simulink model "TV_FLC_V3_Codegen"  (R2026a)
settings: Solver=FixedStepDiscrete  StopTime=100  FixedStep=0.003  MaxStep=0.4  AbsTol=1e-3
model workspace (MAT data in the model file):
  Af = 1.20000004768
  C_alpha_F = 46504
  D = 11
  F = 0.0421790704131
  FIS_DYC_3 : fistree (value not decoded)
  Gain = 0.175131350756
  Gr = 5
  I = 6000
  Kp_TV_Beta = Simulink.Parameter
  Kp_TV_Beta.Value = 600
  Kp_TV_Beta.Complexity = 'real'
  Kp_TV_Beta.Dimensions = [1 1]
  Kp_TV_Beta.CoderInfo.StorageClass = 'ImportedExtern'
  Kp_TV_Beta.DataType = 'single'
  Kp_TV_Yaw = Simulink.Parameter
  Kp_TV_Yaw.Value = 1000
  Kp_TV_Yaw.Complexity = 'real'
  Kp_TV_Yaw.Dimensions = [1 1]
  Kp_TV_Yaw.CoderInfo.StorageClass = 'ImportedExtern'
  Kp_TV_Yaw.DataType = 'single'
  Ku = -0.000124337399029
  L = 1.57799994946
  Load_Ref = [0; 400; 500; 600; 700; 800; 900; 1000; 1100; 1200; 1300; 1400; 1500; 1600; 1700; 1800; 1900; 2000]
  MotorT = [51.0306892395 51.0306892395 51.0306892395 51.0306892395 51.0306892395 51.0306892395 51.0306892395 51.0306892395 51.0306892395 51.0306892395 51.0306892395 51.0306892395 51.0306892395 51.0306892395 51.0306892395 51.0306892395 51.0306892395 51.0306892395 51.0306892395 51.0306892395 51.0306892395 51.0306892395 51.0306892395 51.0306892395 51.0306892395 51.0306892395 51.0306892395 51.0306892395 51.0306892395 51.0306892395 51.0306892395 51.0306892395 51.0306892395 51.0306892395 51.0306892395 51.0306892395 51.0306892395 44.8436889648 36.8215675354 30.0627288818 25.3370742798 21.0374126434 17.0840320587 13.4184885025 9.99592685699 6.7769651413 3.73957490921]
  MotorW = [0 100 200 300 400 500 600 700 800 900 1000 1100 1200 1300 1400 1500 1600 1700 1800 1900 2000 2100 2200 2300 2400 2500 2600 2700 2800 2900 3000 3100 3200 3300 3400 3500 3600 3700 3800 3900 4000 4100 4200 4300 4400 4500 4600]
  P = 800
  Slip_Ctrl_Kd = Simulink.Parameter
  Slip_Ctrl_Kd.Value = 0.5
  Slip_Ctrl_Kd.Complexity = 'real'
  Slip_Ctrl_Kd.Dimensions = [1 1]
  Slip_Ctrl_Kd.CoderInfo.StorageClass = 'ImportedExtern'
  Slip_Ctrl_Kd.DataType = 'single'
  Slip_Ctrl_Ki = Simulink.Parameter
  Slip_Ctrl_Ki.Value = 100
  Slip_Ctrl_Ki.Complexity = 'real'
  Slip_Ctrl_Ki.Dimensions = [1 1]
  Slip_Ctrl_Ki.CoderInfo.StorageClass = 'ImportedExtern'
  Slip_Ctrl_Ki.DataType = 'single'
  Slip_Ctrl_Kn = Simulink.Parameter
  Slip_Ctrl_Kn.Value = 100
  Slip_Ctrl_Kn.Complexity = 'real'
  Slip_Ctrl_Kn.Dimensions = [1 1]
  Slip_Ctrl_Kn.CoderInfo.StorageClass = 'ImportedExtern'
  Slip_Ctrl_Kn.DataType = 'single'
  Slip_Ctrl_Kp = Simulink.Parameter
  Slip_Ctrl_Kp.Value = 90
  Slip_Ctrl_Kp.Complexity = 'real'
  Slip_Ctrl_Kp.Dimensions = [1 1]
  Slip_Ctrl_Kp.CoderInfo.StorageClass = 'ImportedExtern'
  Slip_Ctrl_Kp.DataType = 'single'
  Slip_Ref = [0.151999995112; 0.151999995112; 0.151999995112; 0.115999996662; 0.101999998093; 0.0960000008345; 0.0920000001788; 0.0900000035763; 0.0900000035763; 0.0900000035763; 0.0939999967813; 0.097999997437; 0.104000002146; 0.112000003457; 0.126000002027; 0.153999999166; 0.231999993324; 0.15000000596]
  Slip_Steer_th = Simulink.Parameter
  Slip_Steer_th.Value = 15
  Slip_Steer_th.Complexity = 'real'
  Slip_Steer_th.Dimensions = [1 1]
  Slip_Steer_th.CoderInfo.StorageClass = 'ImportedExtern'
  Slip_Steer_th.DataType = 'single'
  Slip_TC_Enable = Simulink.Parameter
  Slip_TC_Enable.Value = 1
  Slip_TC_Enable.Complexity = 'real'
  Slip_TC_Enable.Dimensions = [1 1]
  Slip_TC_Enable.CoderInfo.StorageClass = 'ImportedExtern'
  Slip_TC_Enable.DataType = 'single'
  Tmax = 51.0306892395
  a = 0.823199987411
  a_cop = 0.707000017166
  cd = -2.15000009537
  g = 9.81000041962
  h_CG = 0.358300000429
  m = 320
  ro = 1.22599995136
  rwheel = 0.263000011444
  tr = 1.24800002575
  vx_th = 1
undefined symbols (not defined in the file or in its folder): dspblkCoreblockFVToolHelper, gcbh
libraries: simulink x5, sl_discontinuities x3, slpidlib x2, fuzblock x1
(part 1 of 2)
settings Model: DataDictionary=TV_FLC_V3_Codegen_BusDefs.sldd  Creator=smiller  LastModifiedBy=andrei
settings SolverCC: MaxConsecutiveMinStep=5  InsertRTBMode=Never (minimum delay)  MinimalZcImpactIntegration=on
settings DataIOCC: SaveFormat=StructureWithTime  SignalLoggingName=logsout_sm_car
settings OptimizationCC: UseDivisionForNetSlopeComputation=on  GainParamInheritBuiltInType=on  UseFloatMulNetSlope=on  DefaultUnderspecifiedDataType=single  UseSpecifiedMinMax=on  NoFixptDivByZeroProtection=on  EfficientFloat2IntCast=on
settings DebuggingCC: ReadBeforeWriteMsg=EnableAllAsError  WriteAfterWriteMsg=EnableAllAsError  WriteAfterReadMsg=EnableAllAsError  IntegerOverflowMsg=error  ParameterPrecisionLossMsg=none  UniqueDataStoreMsg=error  NonBusSignalsTreatedAsBus=error  SFInvalidInputDataAccessInChartInitDiag=error  SFTransitionOutsideNaturalParentDiag=error  SFUnreachableExecutionPathDiag=error  SFUndirectedBroadcastEventsDiag=error  IntegerSaturationMsg=error
settings HardwareCC: ProdLargestAtomicInteger=Long  ProdLargestAtomicFloat=Double  ProdHWDeviceType=ARM Compatible->ARM Cortex-M
settings RTWCC: SystemTargetFile=ert.tlc  BuildConfiguration=Faster Runs  Description=Embedded Coder
settings CodeAppCC: CustomSymbolStrGlobalVar=rt$N_$R$M  CustomSymbolStrType=$N_$R$M  CustomSymbolStrFcn=$N$M$F  CustomSymbolStrMacro=$N$M  CustomSymbolStrUtil=$N_$R$C
settings ERTTargetCC: ERTFilePackagingFormat=CompactWithDataFile  GenerateSampleERTMain=on  IncludeMdlTerminateFcn=off  CombineSignalStateStructs=on  SuppressErrorStatus=on  SupportAbsoluteTime=off  CodeInterfacePackaging=Reusable function  SupportComplex=off
settings SimscapeCC: SimscapeNominalValues="[{\"value\":\"1\",\"unit\":\"A\"},{\"value\":\"1\",\"unit\":\"bar\"},{\"value\":\"1\",\"unit\":\"cm^2\"},{\"value\":\"1\",\"unit\":\"cm^3/s\"},{\"value\":\"1\",\"unit\":\"kJ/kg\"},{\"value\":\"1\",\"unit\":\"kW\"},{\"value\":\"1\",\"unit\":\"l\"},{\"value\":\"1\",\"unit\":\"N\"},{\"value\":\"1\",\"unit\":\"N*m\"},{\"value\":\"1\",\"unit\":\"V\"}]"  SimscapeLogSimulationStatistics=on  SimscapeLogName=simlog_sm_car  SimscapeLogDataHistory=100000.0  SimscapeOperatingPoint=ssc_op
settings DiagnosticsConfigSet: SimMechanicsConflictingReferenceFrames=none  SimMechanicsRigidlyBoundBlock=none  SimMechanicsUnsatisfiedHighPriorityTargets=error
settings ExplorerConfigSet: InternalSimMechanicsExplorerSettings="<ExplorerConfiguration><canonicalview>default</canonicalview><AnimationSetting><BasePlaybackSpeed>1.0</BasePlaybackSpeed><PlaybackSpeedFactor>1.0</PlaybackSpeedFactor></AnimationSetting><TilePanel><TileInfo><Tiles Columns=\"1\" Count=\"1\" Rows=\"1\"><Column Weight=\"1\"/><Row Weight=\"1\"/><Tile Height=\"1\" Width=\"1\" X=\"0\" Y=\"0\"/></Tiles></TileInfo><SceneInfo><SceneViewer><BGColor><R>1</R><G>1</G><B>1</B></BGColor><Camera><DoPerspective>on</DoPerspective><Position><X>-22.5734563329168161</X><Y>-2.56079992530625722</Y><Z>1.4393604008155032</Z></Position><Center><X>-23.2962680852000119</X><Y>-1.95845679840359432</Y><Z>1.10064823948317181</Z></Center><Up><X>-0.260205889993916473</X><Y>0.216838241661597014</Y><Z>0.940890042335224552</Z></Up><ViewLimDist>1</ViewLimDist><YLim>0.466307658154998694</YLim><XLim>0.489818968650208741</XLim></Camera></SceneViewer></SceneInfo></TilePanel><MechEditorPanel><Cameras><Camera><Id>Camera1</Id><Value><Name>Track FixO FR</Name><NativeCamera><PositionTrackingFeature>Camera_Frames.Frame_FixO_FR.R</PositionTrackingFeature><CenterTrackingFeature>Camera_Frames.Frame_FixO_FR.R</CenterTrackingFeature><UpVectorTrackingFeature>Camera_Frames.Frame_FixO_FR.R</UpVectorTrackingFeature><CenterTrackingOrigin>off</CenterTrackingOrigin><CenterTrackingDirection>+X</CenterTrackingDirection><UpVectorTrackingDirection>+Z</UpVectorTrackingDirection></NativeCamera></Value></Camera><Camera><Id>Camera2</Id><Value><Name>Track FixO Right</Name><NativeCamera><PositionTrackingFeature>Camera_Frames.Frame_FixO_Right.R</PositionTrackingFeature><CenterTrackingFeature>Camera_Frames.Transform_Camera_Ref.F</CenterTrackingFeature><UpVectorTrackingFeature>Camera_Frames.Frame_FixO_Right.R</UpVectorTrackingFeature><CenterTrackingOrigin>off</CenterTrackingOrigin><CenterTrackingDirection>+Y</CenterTrackingDirection><UpVectorTrackingDirection>+Z</UpVectorTrackingDirection></NativeCamera></Value></Camera><Camera><Id>Camera3</Id><Value><Name>Track FixO RR</Name><NativeCamera><PositionTrackingFeature>Camera_Frames.Frame_FixO_RR.R</PositionTrackingFeature><CenterTrackingFeature>Camera_Frames.Frame_FixO_RR.R</CenterTrackingFeature><UpVectorTrackingFeature>Camera_Frames.Frame_FixO_RR.R</UpVectorTrackingFeature><CenterTrackingOrigin>off</CenterTrackingOrigin><CenterTrackingDirection>+X</CenterTrackingDirection><UpVectorTrackingDirection>+Z</UpVectorTrackingDirection></NativeCamera></Value></Camera><Camera><Id>Camera4</Id><Value><Name>Track FixO RL</Name><NativeCamera><PositionTrackingFeature>Camera_Frames.Frame_FixO_RL.R</PositionTrackingFeature><CenterTrackingFeature>Camera_Frames.Frame_FixO_RL.R</CenterTrackingFeature><UpVectorTrackingFeature>Camera_Frames.Frame_FixO_RL.R</UpVectorTrackingFeature><CenterTrackingOrigin>off</CenterTrackingOrigin><CenterTrackingDirection>+X</CenterTrackingDirection><UpVectorTrackingDirection>+Z</UpVectorTrackingDirection></NativeCamera></Value></Camera><Camera><Id>Camera5</Id><Value><Name>Track FixO Left</Name><NativeCamera><PositionTrackingFeature>Camera_Frames.Frame_FixO_Left.R</PositionTrackingFeature><CenterTrackingFeature>Camera_Frames.Transform_Camera_Ref.F</CenterTrackingFeature><UpVectorTrackingFeature>Camera_Frames.Frame_FixO_Left.R</UpVectorTrackingFeature><CenterTrackingOrigin>off</CenterTrackingOrigin><CenterTrackingDirection>-Y</CenterTrackingDirection><UpVectorTrackingDirection>+Z</UpVectorTrackingDirection></NativeCamera></Value></Camera><Camera><Id>Camera6</Id><Value><Name>Track FixO FL</Name><NativeCamera><PositionTrackingFeature>Camera_Frames.Frame_FixO_FL.R</PositionTrackingFeature><CenterTrackingFeature>Camera_Frames.Frame_FixO_FL.R</CenterTrackingFeature><UpVectorTrackingFeature>Camera_Frames.Frame_FixO_FL.R</UpVectorTrackingFeature><CenterTrackingOrigin>off</CenterTrackingOrigin><CenterTrackingDirection>+X</CenterTrackingDirection><UpVectorTrackingDirection>+Z</UpVectorTrackingDirection></NativeCamera></Value></Camera><Camera><Id>Camera7</Id><Value><Name>Track FixO Top</Name><NativeCamera><PositionTrackingFeature>Camera_Frames.Frame_FixO_Top.R</PositionTrackingFeature><CenterTrackingFeature>Camera_Frames.Frame_FixO_Top.R</CenterTrackingFeature><UpVectorTrackingFeature>Camera_Frames.Frame_FixO_Top.R</UpVectorTrackingFeature><CenterTrackingOrigin>off</CenterTrackingOrigin><CenterTrackingDirection>+X</CenterTrackingDirection><UpVectorTrackingDirection>+Z</UpVectorTrackingDirection></NativeCamera></Value></Camera><Camera><Id>Camera8</Id><Value><Name>Track FixO Front</Name><NativeCamera><PositionTrackingFeature>Camera_Frames.Frame_FixO_Front.R</PositionTrackingFeature><CenterTrackingFeature>Camera_Frames.Frame_FixO_Front.R</CenterTrackingFeature><UpVectorTrackingFeature>Camera_Frames.Frame_FixO_Front.R</UpVectorTrackingFeature><CenterTrackingOrigin>off</CenterTrackingOrigin><CenterTrackingDirection>+X</CenterTrackingDirection><UpVectorTrackingDirection>+Z</UpVectorTrackingDirection></NativeCamera></Value></Camera><Camera><Id>Camera9</Id><Value><Name>Track FixO Rear</Name><NativeCamera><PositionTrackingFeature>Camera_Frames.Frame_FixO_Rear.R</PositionTrackingFeature><CenterTrackingFeature>Camera_Frames.Frame_FixO_Rear.R</CenterTrackingFeature><UpVectorTrackingFeature>Camera_Frames.Frame_FixO_Rear.R</UpVectorTrackingFeature><CenterTrackingOrigin>off</CenterTrackingOrigin><CenterTrackingDirection>+X</CenterTrackingDirection><UpVectorTrackingDirection>+Z</UpVectorTrackingDirection></NativeCamera></Value></Camera><Camera><Id>Camera10</Id><Value><Name>Track FR</Name><NativeCamera><PositionTrackingFeature>Camera_Frames.Frame_FR.R</PositionTrackingFeature><CenterTrackingFeature>Camera_Frames.Frame_FR.R</CenterTrackingFeature><UpVectorTrackingFeature>Camera_Frames.Frame_FR.R</UpVectorTrackingFeature><CenterTrackingOrigin>off</CenterTrackingOrigin><CenterTrackingDirection>+X</CenterTrackingDirection><UpVectorTrackingDirection>+Z</UpVectorTrackingDirection></NativeCamera></Value></Camera><Camera><Id>Camera11</Id><Value><Name>Track Right</Name><NativeCamera><PositionTrackingFeature>Camera_Frames.Frame_Right.R</PositionTrackingFeature><CenterTrackingFeature>Camera_Frames.Transform_Camera_Ref.F</CenterTrackingFeature><UpVectorTrackingFeature>Camera_Frames.Frame_Right.R</UpVectorTrackingFeature><CenterTrackingOrigin>off</CenterTrackingOrigin><CenterTrackingDirection>+Y</CenterTrackingDirection><UpVectorTrackingDirection>+Z</UpVectorTrackingDirection></NativeCamera></Value></Camera><Camera><Id>Camera12</Id><Value><Name>Track RR</Name><NativeCamera><PositionTrackingFeature>Camera_Frames.Frame_RR.R</PositionTrackingFeature><CenterTrackingFeature>Camera_Frames.Frame_RR.R</CenterTrackingFeature><UpVectorTrackingFeature>Camera_Frames.Frame_RR.R</UpVectorTrackingFeature><CenterTrackingOrigin>off</CenterTrackingOrigin><CenterTrackingDirection>+X</CenterTrackingDirection><UpVectorTrackingDirection>+Z</UpVectorTrackingDirection></NativeCamera></Value></Camera><Camera><Id>Camera13</Id><Value><Name>Track RL</Name><NativeCamera><PositionTrackingFeature>Camera_Frames.Frame_RL.R</PositionTrackingFeature><CenterTrackingFeature>Camera_Frames.Frame_RL.R</CenterTrackingFeature><UpVectorTrackingFeature>Camera_Frames.Frame_RL.R</UpVectorTrackingFeature><CenterTrackingOrigin>off</CenterTrackingOrigin><CenterTrackingDirection>+X</CenterTrackingDirection><UpVectorTrackingDirection>+Z</UpVectorTrackingDirection></NativeCamera></Value></Camera><Camera><Id>Camera14</Id><Value><Name>Track Left</Name><NativeCamera><PositionTrackingFeature>Camera_Frames.Frame_Left.R</PositionTrackingFeature><CenterTrackingFeature>Camera_Frames.Transform_Camera_Ref.F</CenterTrackingFeature><UpVectorTrackingFeature>Camera_Frames.Frame_Left.R</UpVectorTrackingFeature><CenterTrackingOrigin>off</CenterTrackingOrigin><CenterTrackingDirection>-Y</CenterTrackingDirection><UpVectorTrackingDirection>+Z</UpVectorTrackingDirection></NativeCamera></Value></Camera><Camera><Id>Camera15</Id><Value><Name>Track FL</Name><NativeCamera><PositionTrackingFeature>Camera_Frames.Frame_FL.R</PositionTrackingFeature><CenterTrackingFeature>Camera_Frames.Frame_FL.R</CenterTrackingFeature><UpVectorTrackingFeature>Camera_Frames.Frame_FL.R</UpVectorTrackingFeature><CenterTrackingOrigin>off</CenterTrackingOrigin><CenterTrackingDirection>+X</CenterTrackingDirection><UpVectorTrackingDirection>+Z</UpVectorTrackingDirection></NativeCamera></Value></Camera><Camera><Id>Camera16</Id><Value><Name>Track Top</Name><NativeCamera><PositionTrackingFeature>Camera_Frames.Frame_Top.R</PositionTrackingFeature><CenterTrackingFeature>Camera_Frames.Frame_Top.R</CenterTrackingFeature><UpVectorTrackingFeature>Camera_Frames.Frame_Top.R</UpVectorTrackingFeature><CenterTrackingOrigin>off</CenterTrackingOrigin><CenterTrackingDirection>+X</CenterTrackingDirection><UpVectorTrackingDirection>+Z</UpVectorTrackingDirection></NativeCamera></Value></Camera><Camera><Id>Camera17</Id><Value><Name>Track Front</Name><NativeCamera><PositionTrackingFeature>Camera_Frames.Frame_Front.R</PositionTrackingFeature><CenterTrackingFeature>Camera_Frames.Frame_Front.R</CenterTrackingFeature><UpVectorTrackingFeature>Camera_Frames.Frame_Front.R</UpVectorTrackingFeature><CenterTrackingOrigin>off</CenterTrackingOrigin><CenterTrackingDirection>+X</CenterTrackingDirection><UpVectorTrackingDirection>+Z</UpVectorTrackingDirection></NativeCamera></Value></Camera><Camera><Id>Camera18</Id><Value><Name>Track Rear</Name><NativeCamera><PositionTrackingFeature>Camera_Frames.Frame_Rear.R</PositionTrackingFeature><CenterTrackingFeature>Camera_Frames.Frame_Rear.R</CenterTrackingFeature><UpVectorTrackingFeature>Camera_Frames.Frame_Rear.R</UpVectorTrackingFeature><CenterTrackingOrigin>off</CenterTrackingOrigin><CenterTrackingDirection>+X</CenterTrackingDirection><UpVectorTrackingDirection>+Z</UpVectorTrackingDirection></NativeCamera></Value></Camera><Camera><Id>Camera19</Id><Value><Name>Track SuspF</Name><NativeCamera><PositionTrackingFeature>Camera_Frames.Frame_SuspF.R</PositionTrackingFeature><CenterTrackingFeature>Camera_Frames.Frame_SuspF.R</CenterTrackingFeature><UpVectorTrackingFeature>Camera_Frames.Frame_SuspF.R</UpVectorTrackingFeature><CenterTrackingOrigin>off</CenterTrackingOrigin><CenterTrackingDirection>+X</CenterTrackingDirection><UpVectorTrackingDirection>+Z</UpVectorTrackingDirection></NativeCamera></Value></Camera><Camera><Id>Camera20</Id><Value><Name>Track SuspR</Name><NativeCamera><PositionTrackingFeature>Camera_Frames.Frame_SuspR.R</PositionTrackingFeature><CenterTrackingFeature>Camera_Frames.Frame_SuspR.R</CenterTrackingFeature><UpVectorTrackingFeature>Camera_Frames.Frame_SuspR.R</UpVectorTrackingFeature><CenterTrackingOrigin>off</CenterTrackingOrigin><CenterTrackingDirection>+X</CenterTrackingDirection><UpVectorTrackingDirection>+Z</UpVectorTrackingDirection></NativeCamera></Value></Camera><Camera><Id>Camera21</Id><Value><Name>Track WheelFR</Name><NativeCamera><PositionTrackingFeature>Camera_Frames.Frame_Wheel_FR.R</PositionTrackingFeature><CenterTrackingFeature>Camera_Frames.Frame_Wheel_FR.R</CenterTrackingFeature><UpVectorTrackingFeature>Camera_Frames.Frame_Wheel_FR.R</UpVectorTrackingFeature><CenterTrackingOrigin>off</CenterTrackingOrigin><CenterTrackingDirection>+X</CenterTrackingDirection><UpVectorTrackingDirection>+Z</UpVectorTrackingDirection></NativeCamera></Value></Camera><Camera><Id>Camera22</Id><Value><Name>Track WheelRR</Name><NativeCamera><PositionTrackingFeature>Camera_Frames.Frame_Wheel_RR.R</PositionTrackingFeature><CenterTrackingFeature>Camera_Frames.Frame_Wheel_RR.R</CenterTrackingFeature><UpVectorTrackingFeature>Camera_Frames.Frame_Wheel_RR.R</UpVectorTrackingFeature><CenterTrackingOrigin>off</CenterTrackingOrigin><CenterTrackingDirection>+X</CenterTrackingDirection><UpVectorTrackingDirection>+Z</UpVectorTrackingDirection></NativeCamera></Value></Camera><Camera><Id>Camera23</Id><Value><Name>Track WheelRL</Name><NativeCamera><PositionTrackingFeature>Camera_Frames.Frame_Wheel_RL.R</PositionTrackingFeature><CenterTrackingFeature>Camera_Frames.Frame_Wheel_RL.R</CenterTrackingFeature><UpVectorTrackingFeature>Camera_Frames.Frame_Wheel_RL.R</UpVectorTrackingFeature><CenterTrackingOrigin>off</CenterTrackingOrigin><CenterTrackingDirection>+X</CenterTrackingDirection><UpVectorTrackingDirection>+Z</UpVectorTrackingDirection></NativeCamera></Value></Camera><Camera><Id>Camera24</Id><Value><Name>Track WheelFL</Name><NativeCamera><PositionTrackingFeature>Camera_Frames.Frame_Wheel_FL.R</PositionTrackingFeature><CenterTrackingFeature>Camera_Frames.Frame_Wheel_FL.R</CenterTrackingFeature><UpVectorTrackingFeature>Camera_Frames.Frame_Wheel_FL.R</UpVectorTrackingFeature><CenterTrackingOrigin>off</CenterTrackingOrigin><CenterTrackingDirection>+X</CenterTrackingDirection><UpVectorTrackingDirection>+Z</UpVectorTrackingDirection></NativeCamera></Value></Camera><Camera><Id>Camera25</Id><Value><Name>View Seat FL</Name><NativeCamera><PositionTrackingFeature>Camera_Frames.Frame_View_Seat_FL.R</PositionTrackingFeature><CenterTrackingFeature>Camera_Frames.Frame_View_Seat_FL.R</CenterTrackingFeature><UpVectorTrackingFeature>Camera_Frames.Frame_View_Seat_FL.R</UpVectorTrackingFeature><CenterTrackingOrigin>off</CenterTrackingOrigin><CenterTrackingDirection>+X</CenterTrackingDirection><UpVectorTrackingDirection>+Z</UpVectorTrackingDirection></NativeCamera></Value></Camera><Camera><Id>Camera26</Id><Value><Name>View Seat FR</Name><NativeCamera><PositionTrackingFeature>Camera_Frames.Frame_View_Seat_FR.R</PositionTrackingFeature><CenterTrackingFeature>Camera_Frames.Frame_View_Seat_FR.R</CenterTrackingFeature><UpVectorTrackingFeature>Camera_Frames.Frame_View_Seat_FR.R</UpVectorTrackingFeature><CenterTrackingOrigin>off</CenterTrackingOrigin><CenterTrackingDirection>+X</CenterTrackingDirection><UpVectorTrackingDirection>+Z</UpVectorTrackingDirection></NativeCamera></Value></Camera><Camera><Id>Camera27</Id><Value><Name>View Susp FR</Name><NativeCamera><PositionTrackingFeature>Camera_Frames.Frame_View_Susp_FR.R</PositionTrackingFeature><CenterTrackingFeature>Camera_Frames.Frame_View_Susp_FR.R</CenterTrackingFeature><UpVectorTrackingFeature>Camera_Frames.Frame_View_Susp_FR.R</UpVectorTrackingFeature><CenterTrackingOrigin>off</CenterTrackingOrigin><CenterTrackingDirection>+X</CenterTrackingDirection><UpVectorTrackingDirection>+Z</UpVectorTrackingDirection></NativeCamera></Value></Camera><Camera><Id>Camera28</Id><Value><Name>View Susp RR</Name><NativeCamera><PositionTrackingFeature>Camera_Frames.Frame_View_Susp_RR.R</PositionTrackingFeature><CenterTrackingFeature>Camera_Frames.Frame_View_Susp_RR.R</CenterTrackingFeature><UpVectorTrackingFeature>Camera_Frames.Frame_View_Susp_RR.R</UpVectorTrackingFeature><CenterTrackingOrigin>off</CenterTrackingOrigin><CenterTrackingDirection>+X</CenterTrackingDirection><UpVectorTrackingDirection>+Z</UpVectorTrackingDirection></NativeCamera></Value></Camera><Camera><Id>Camera29</Id><Value><Name>View Susp RL</Name><NativeCamera><PositionTrackingFeature>Camera_Frames.Frame_View_Susp_RL.R</PositionTrackingFeature><CenterTrackingFeature>Camera_Frames.Frame_View_Susp_RL.R</CenterTrackingFeature><UpVectorTrackingFeature>Camera_Frames.Frame_View_Susp_RL.R</UpVectorTrackingFeature><CenterTrackingOrigin>off</CenterTrackingOrigin><CenterTrackingDirection>+X</CenterTrackingDirection><UpVectorTrackingDirection>+Z</UpVectorTrackingDirection></NativeCamera></Value></Camera><Camera><Id>Camera30</Id><Value><Name>View Susp FL</Name><NativeCamera><PositionTrackingFeature>Camera_Frames.Frame_View_Susp_FL.R</PositionTrackingFeature><CenterTrackingFeature>Camera_Frames.Frame_View_Susp_FL.R</CenterTrackingFeature><UpVectorTrackingFeature>Camera_Frames.Frame_View_Susp_FL.R</UpVectorTrackingFeature><CenterTrackingOrigin>off</CenterTrackingOrigin><CenterTrackingDirection>+X</CenterTrackingDirection><UpVectorTrackingDirection>+Z</UpVectorTrackingDirection></NativeCamera></Value></Camera><Camera><Id>Camera31</Id><Value><Name>Dolly Camera</Name><NativeCamera><PositionTrackingFeature>Camera_Frames.Frame_Dolly.R</PositionTrackingFeature><CenterTrackingFeature>Camera_Frames.Frame_Dolly.R</CenterTrackingFeature><UpVectorTrackingFeature>Camera_Frames.Frame_Dolly.R</UpVectorTrackingFeature><CenterTrackingOrigin>off</CenterTrackingOrigin><CenterTrackingDirection>+X</CenterTrackingDirection><UpVectorTrackingDirection>+Z</UpVectorTrackingDirection></NativeCamera></Value></Camera><Camera><Id>Camera32</Id><Value><Name>Track Dolly Camera</Name><NativeCamera><PositionTrackingFeature>Camera_Frames.Frame_Dolly.R</PositionTrackingFeature><CenterTrackingFeature>Camera_Frames.Transform_Camera_Ref.F</CenterTrackingFeature><UpVectorTrackingFeature>Camera_Frames.World_Frame.W</UpVectorTrackingFeature><CenterTrackingOrigin>on</CenterTrackingOrigin><UpVectorTrackingDirection>+Z</UpVectorTrackingDirection></NativeCamera></Value></Camera></Cameras><GfxPanelCameraMap><MapElement CameraMLId=\"Camera1\" GfxPanelIndex=\"0\"/></GfxPanelCameraMap><VideoCreator><PlaybackSpeedRatio>1.0</PlaybackSpeedRatio><FrameRate>30</FrameRate><VideoFormat>MPEG-4</VideoFormat><FrameSize>[800 450]</FrameSize></VideoCreator></MechEditorPanel></ExplorerConfiguration>"

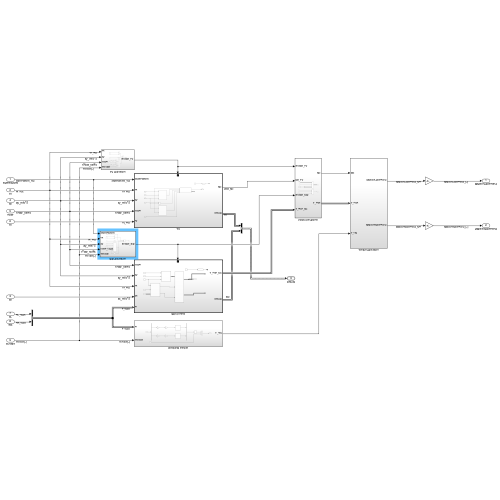
[thumbnail: Simulink's stored preview of the top-level diagram]
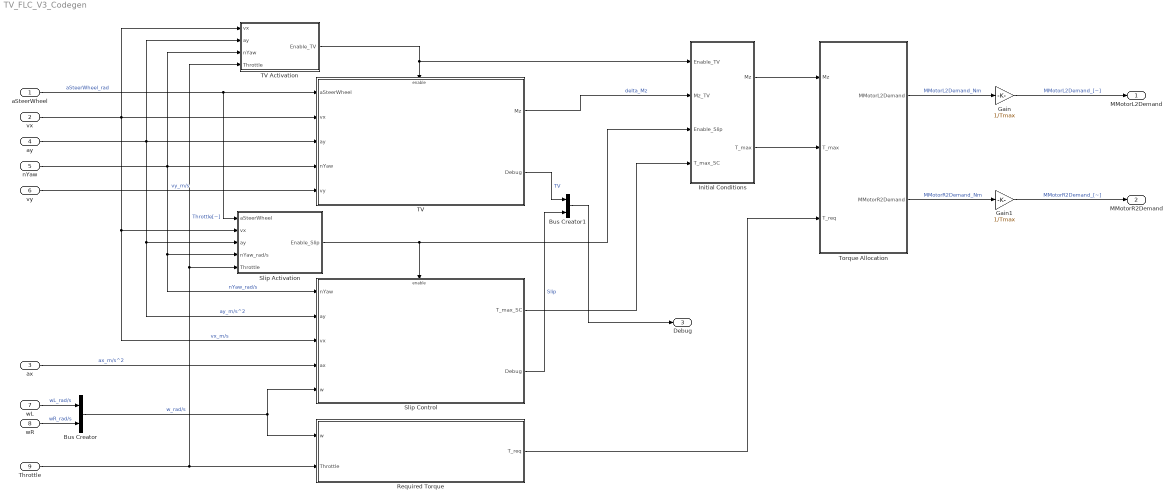
== system TV_FLC_V3_Codegen ==
  aSteerWheel : Inport  OutDataTypeStr=single  PortDimensions=1  SampleTime=0.003
  vx : Inport  Port=2  OutDataTypeStr=single  PortDimensions=1  SampleTime=0.003
  ax : Inport  Port=3  OutDataTypeStr=single  PortDimensions=1  SampleTime=0.003
  ay : Inport  Port=4  OutDataTypeStr=single  PortDimensions=1  SampleTime=0.003
  nYaw : Inport  Port=5  OutDataTypeStr=single  PortDimensions=1  SampleTime=0.003
  vy : Inport  Port=6  OutDataTypeStr=single  PortDimensions=1  SampleTime=0.003
  wL : Inport  Port=7  OutDataTypeStr=single  PortDimensions=1  SampleTime=0.003
  wR : Inport  Port=8  OutDataTypeStr=single  PortDimensions=1  SampleTime=0.003
  Throttle : Inport  Port=9  OutDataTypeStr=single  PortDimensions=1  SampleTime=0.003
  Bus Creator : BusCreator  Inputs=2
  Bus Creator1 : BusCreator  Inputs=2  OutDataTypeStr=Bus: Debug  NonVirtualBus=on
  Gain : Gain  Gain=1/Tmax
  Gain1 : Gain  Gain=1/Tmax
  Initial Conditions : Subsystem
  Required Torque : Subsystem
  Slip Activation : Subsystem
  Slip Control : Subsystem
  TV : Subsystem
  TV Activation : Subsystem
  Torque Allocation : Subsystem
  MMotorL2Demand : Outport  OutDataTypeStr=single  PortDimensions=1  SampleTime=0.003
  MMotorR2Demand : Outport  Port=2  OutDataTypeStr=single  PortDimensions=1  SampleTime=0.003
  Debug : Outport  Port=3  OutDataTypeStr=Bus: Debug  SampleTime=0.003
  wires:
  vy/1 -> TV/5(vy)  "vy_m/s"
  aSteerWheel/1 -> TV/1(aSteerWheel), Slip Activation/1(aSteerWheel)  "aSteerWheel_rad"
  TV/2(Debug) -> Bus Creator1/1  "TV"
  Required Torque/1(T_req) -> Torque Allocation/3(T_req)
  wR/1 -> Bus Creator/2  "wR_rad/s"
  Gain1/1 -> MMotorR2Demand/1  "MMotorR2Demand_[~]"
  TV Activation/1(Enable_TV) -> TV/Enable, Initial Conditions/1(Enable_TV)
  vx/1 -> TV/2(vx), Slip Control/3(vx), Slip Activation/2(vx), TV Activation/1(vx)  "vx_m/s"
  Slip Activation/1(Enable_Slip) -> Initial Conditions/3(Enable_Slip), Slip Control/Enable
  Initial Conditions/2(T_max) -> Torque Allocation/2(T_max)
  ax/1 -> Slip Control/4(ax)  "ax_m/s^2"
  Gain/1 -> MMotorL2Demand/1  "MMotorL2Demand_[~]"
  Slip Control/1(T_max_SC) -> Initial Conditions/4(T_max_SC)
  TV/1(Mz) -> Initial Conditions/2(Mz_TV)  "delta_Mz"
  ay/1 -> TV/3(ay), TV Activation/2(ay), Slip Control/2(ay), Slip Activation/3(ay)  "ay_m/s^2"
  Slip Control/2(Debug) -> Bus Creator1/2  "Slip"
  Initial Conditions/1(Mz) -> Torque Allocation/1(Mz)
  Torque Allocation/1(MMotorL2Demand) -> Gain/1  "MMotorL2Demand_Nm"
  wL/1 -> Bus Creator/1  "wL_rad/s"
  Torque Allocation/2(MMotorR2Demand) -> Gain1/1  "MMotorR2Demand_Nm"
  Bus Creator/1 -> Slip Control/5(w), Required Torque/1(w)  "w_rad/s"
  nYaw/1 -> Slip Control/1(nYaw), Slip Activation/4(nYaw_rad/s), TV/4(nYaw), TV Activation/3(nYaw)  "nYaw_rad/s"
  Throttle/1 -> Required Torque/2(Throttle), Slip Activation/5(Throttle), TV Activation/4(Throttle)  "Throttle[~]"
  Bus Creator1/1 -> Debug/1

== system TV_FLC_V3_Codegen/Initial Conditions ==
  Enable_TV : Inport
  Mz_TV : Inport  Port=2
  Enable_Slip : Inport  Port=3
  T_max_SC : Inport  Port=4
  Bus Creator1 : BusCreator  Inputs=2
  Constant : Constant  Value=Tmax  OutDataTypeStr=single
  Constant1 : Constant  Value=Tmax  OutDataTypeStr=single
  Constant2 : Constant  Value=0  OutDataTypeStr=single
  Switch : Switch  Criteria=u2 ~= 0  SaturateOnIntegerOverflow=off  InputSameDT=off
  Switch1 : Switch  Criteria=u2 ~= 0  SaturateOnIntegerOverflow=off  InputSameDT=off
  Mz : Outport
  T_max : Outport  Port=2
  wires:
  Switch1/1 -> Mz/1
  Constant2/1 -> Switch1/3  "Mz"
  Mz_TV/1 -> Switch1/1
  Constant/1 -> Bus Creator1/1  "Tmax_rl_Nm"
  T_max_SC/1 -> Switch/1
  Bus Creator1/1 -> Switch/3
  Switch/1 -> T_max/1
  Constant1/1 -> Bus Creator1/2  "Tmax_rr_Nm"
  Enable_TV/1 -> Switch1/2
  Enable_Slip/1 -> Switch/2

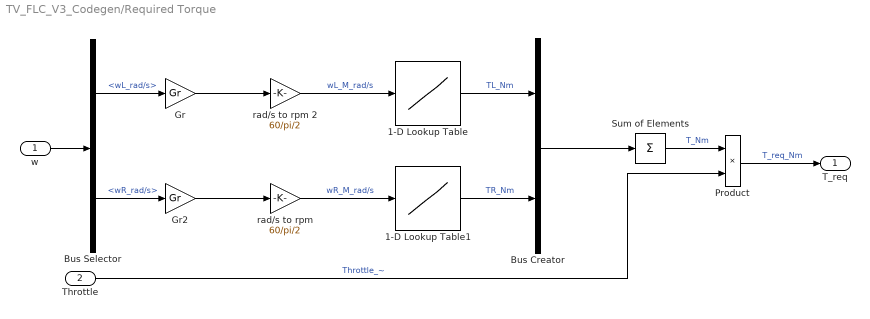
== system TV_FLC_V3_Codegen/Required Torque ==
  w : Inport
  Throttle : Inport  Port=2
  1-D Lookup Table : Lookup_n-D  NumberOfTableDimensions=1  BreakpointsForDimension1=MotorW  Table=MotorT  InternalRulePriority=Speed  RndMeth=Simplest
  1-D Lookup Table1 : Lookup_n-D  NumberOfTableDimensions=1  BreakpointsForDimension1=MotorW  Table=MotorT  InternalRulePriority=Speed  RndMeth=Simplest
  Bus Creator : BusCreator  Inputs=2
  Bus Selector : BusSelector  OutputSignals=wL_rad/s,wR_rad/s
  Gr : Gain  Gain=Gr
  Gr2 : Gain  Gain=Gr
  Product : Product
  Sum of Elements : Sum  Inputs=+
  rad/s to rpm : Gain  Gain=60/pi/2
  rad/s to rpm 2 : Gain  Gain=60/pi/2
  T_req : Outport
  wires:
  Gr2/1 -> rad/s to rpm/1
  Gr/1 -> rad/s to rpm 2/1
  Bus Creator/1 -> Sum of Elements/1
  1-D Lookup Table/1 -> Bus Creator/1  "TL_Nm"
  rad/s to rpm 2/1 -> 1-D Lookup Table/1  "wL_M_rad/s"
  Bus Selector/2 -> Gr2/1  "<wR_rad/s>"
  Product/1 -> T_req/1  "T_req_Nm"
  Bus Selector/1 -> Gr/1  "<wL_rad/s>"
  rad/s to rpm/1 -> 1-D Lookup Table1/1  "wR_M_rad/s"
  Throttle/1 -> Product/2  "Throttle_~"
  1-D Lookup Table1/1 -> Bus Creator/2  "TR_Nm"
  Sum of Elements/1 -> Product/1  "T_Nm"
  w/1 -> Bus Selector/1

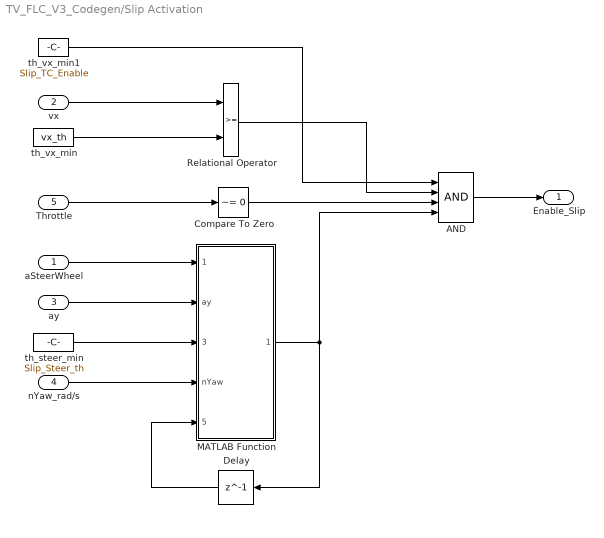
== system TV_FLC_V3_Codegen/Slip Activation ==
  aSteerWheel : Inport
  vx : Inport  Port=2
  ay : Inport  Port=3
  nYaw_rad/s : Inport  Port=4
  Throttle : Inport  Port=5
  AND : Logic  Inputs=4  AllPortsSameDT=off  OutDataTypeStr=boolean
  Compare To Zero : simulink/Logic and Bit Operations/Compare To Zero  relop=~=  OutDataTypeStr=boolean
  Delay : Delay  DelayLength=1
  MATLAB Function : MATLAB Function  TreatAsAtomicUnit=on
  Relational Operator : RelationalOperator  OutDataTypeStr=boolean  RndMeth=Simplest  InputSameDT=off
  th_steer_min : Constant  Value=Slip_Steer_th
  th_vx_min : Constant  Value=vx_th
  th_vx_min1 : Constant  Value=Slip_TC_Enable
  Enable_Slip : Outport
  wires:
  Delay/1 -> MATLAB Function/5(slip_active_previous)
  MATLAB Function/1(slip_active) -> AND/4, Delay/1
  nYaw_rad/s/1 -> MATLAB Function/4(nYaw)
  ay/1 -> MATLAB Function/2(ay)
  th_steer_min/1 -> MATLAB Function/3(steer_th)
  aSteerWheel/1 -> MATLAB Function/1(aSteerWheel)
  Relational Operator/1 -> AND/2
  vx/1 -> Relational Operator/1
  th_vx_min/1 -> Relational Operator/2
  Throttle/1 -> Compare To Zero/1
  AND/1 -> Enable_Slip/1
  Compare To Zero/1 -> AND/3
  th_vx_min1/1 -> AND/1

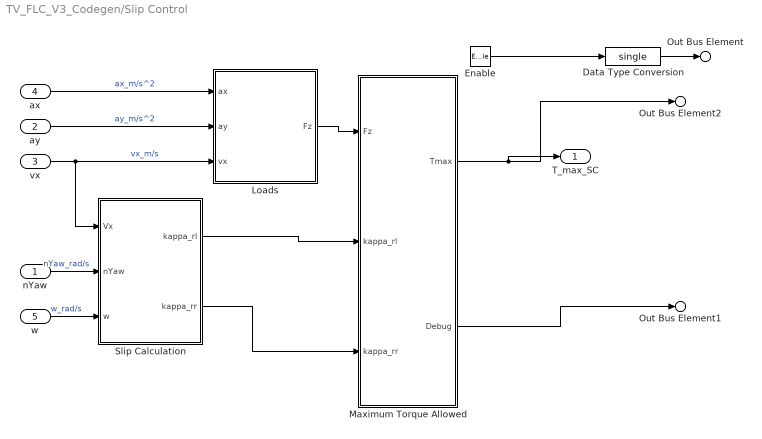
== system TV_FLC_V3_Codegen/Slip Control ==
  nYaw : Inport
  ay : Inport  Port=2
  vx : Inport  Port=3
  ax : Inport  Port=4
  w : Inport  Port=5
  Enable : EnablePort  StatesWhenEnabling=reset  ShowOutputPort=on  OutDataTypeStr=boolean
  Data Type Conversion : DataTypeConversion  OutDataTypeStr=single  SaturateOnIntegerOverflow=off  RndMeth=Floor
  Loads : Subsystem
  Maximum Torque Allowed : Subsystem
  Slip Calculation : Subsystem
  T_max_SC : Outport  OutputWhenDisabled=reset  InitialOutput=Tmax
  Out Bus Element : Outport  Port=2  PortName=Debug  Element=State
  Out Bus Element1 : Outport  Port=2  PortName=Debug  Element=Controller
  Out Bus Element2 : Outport  Port=2  PortName=Debug  Element=TmaxOut
  wires:
  Maximum Torque Allowed/1(Tmax) -> T_max_SC/1, Out Bus Element2/1
  Data Type Conversion/1 -> Out Bus Element/1
  Slip Calculation/1(kappa_rl) -> Maximum Torque Allowed/2(kappa_rl)
  vx/1 -> Slip Calculation/1(Vx), Loads/3(vx)  "vx_m/s"
  Slip Calculation/2(kappa_rr) -> Maximum Torque Allowed/3(kappa_rr)
  ay/1 -> Loads/2(ay)  "ay_m/s^2"
  Loads/1(Fz) -> Maximum Torque Allowed/1(Fz)
  ax/1 -> Loads/1(ax)  "ax_m/s^2"
  nYaw/1 -> Slip Calculation/2(nYaw)  "nYaw_rad/s"
  w/1 -> Slip Calculation/3(w)  "w_rad/s"
  Enable/1 -> Data Type Conversion/1
  Maximum Torque Allowed/2(Debug) -> Out Bus Element1/1

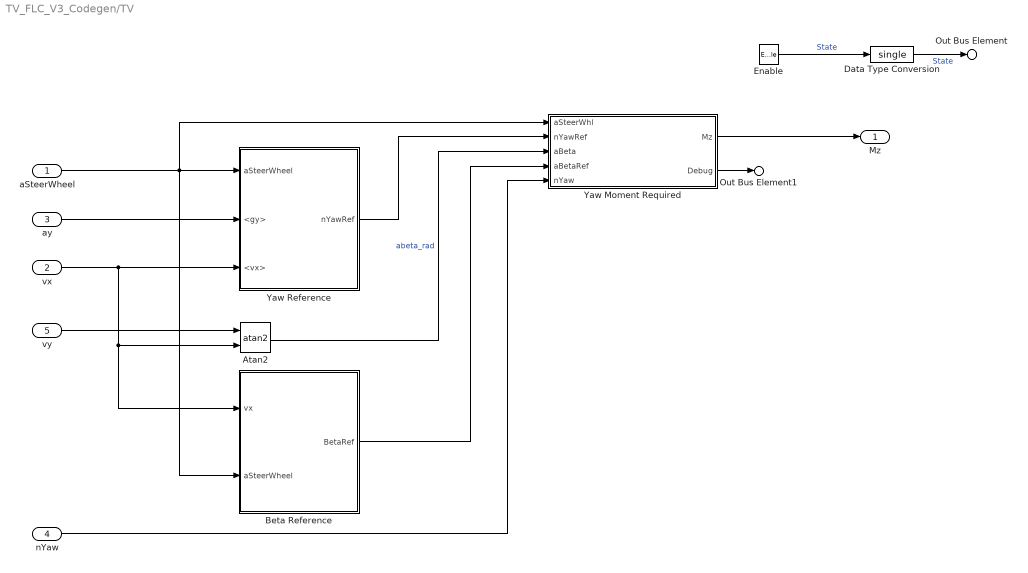
== system TV_FLC_V3_Codegen/TV ==
  aSteerWheel : Inport
  vx : Inport  Port=2
  ay : Inport  Port=3
  nYaw : Inport  Port=4
  vy : Inport  Port=5
  Enable : EnablePort  StatesWhenEnabling=reset  ShowOutputPort=on  OutDataTypeStr=boolean
  Atan2 : Trigonometry  Operator=atan2
  Beta Reference : Subsystem
  Data Type Conversion : DataTypeConversion  OutDataTypeStr=single  SaturateOnIntegerOverflow=off  RndMeth=Floor
  Yaw Moment Required : Subsystem
  Yaw Reference : Subsystem
  Mz : Outport  OutputWhenDisabled=reset  InitialOutput=0
  Out Bus Element : Outport  Port=2  PortName=Debug  Element=State
  Out Bus Element1 : Outport  Port=2  PortName=Debug  Element=Controller
  wires:
  Enable/1 -> Data Type Conversion/1  "State"
  Yaw Moment Required/1(Mz) -> Mz/1
  Atan2/1 -> Yaw Moment Required/3(aBeta)  "abeta_rad"
  aSteerWheel/1 -> Beta Reference/2(aSteerWheel), Yaw Moment Required/1(aSteerWhl), Yaw Reference/1(aSteerWheel)
  vx/1 -> Beta Reference/1(vx), Atan2/2, Yaw Reference/3(<vx>)
  nYaw/1 -> Yaw Moment Required/5(nYaw)
  ay/1 -> Yaw Reference/2(<gy>)
  Yaw Reference/1(nYawRef) -> Yaw Moment Required/2(nYawRef)
  Beta Reference/1(BetaRef) -> Yaw Moment Required/4(aBetaRef)
  vy/1 -> Atan2/1
  Data Type Conversion/1 -> Out Bus Element/1  "State"
  Yaw Moment Required/2(Debug) -> Out Bus Element1/1

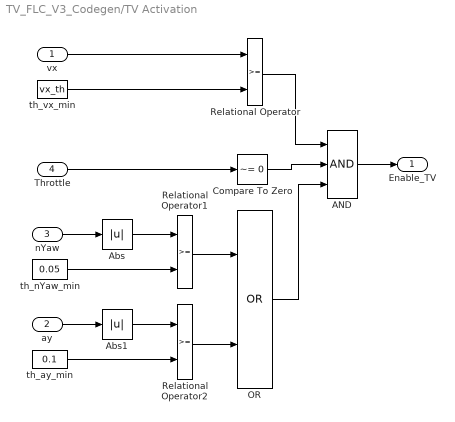
== system TV_FLC_V3_Codegen/TV Activation ==
  vx : Inport
  ay : Inport  Port=2
  nYaw : Inport  Port=3
  Throttle : Inport  Port=4
  AND : Logic  Inputs=3  AllPortsSameDT=off  OutDataTypeStr=boolean
  Abs : Abs  SaturateOnIntegerOverflow=off
  Abs1 : Abs  SaturateOnIntegerOverflow=off
  Compare To Zero : simulink/Logic and Bit Operations/Compare To Zero  relop=~=  OutDataTypeStr=boolean
  OR : Logic  Operator=OR  AllPortsSameDT=off  OutDataTypeStr=boolean
  Relational Operator : RelationalOperator  OutDataTypeStr=boolean  RndMeth=Simplest  InputSameDT=off
  Relational Operator1 : RelationalOperator  OutDataTypeStr=boolean  RndMeth=Simplest  InputSameDT=off
  Relational Operator2 : RelationalOperator  OutDataTypeStr=boolean  RndMeth=Simplest  InputSameDT=off
  th_ay_min : Constant  Value=0.1  OutDataTypeStr=single
  th_nYaw_min : Constant  Value=0.05  OutDataTypeStr=single
  th_vx_min : Constant  Value=vx_th
  Enable_TV : Outport
  wires:
  AND/1 -> Enable_TV/1
  OR/1 -> AND/3
  Compare To Zero/1 -> AND/2
  Relational Operator/1 -> AND/1
  Relational Operator2/1 -> OR/2
  Relational Operator1/1 -> OR/1
  th_vx_min/1 -> Relational Operator/2
  th_ay_min/1 -> Relational Operator2/2
  nYaw/1 -> Abs/1
  vx/1 -> Relational Operator/1
  Abs/1 -> Relational Operator1/1
  Throttle/1 -> Compare To Zero/1
  Abs1/1 -> Relational Operator2/1
  th_nYaw_min/1 -> Relational Operator1/2
  ay/1 -> Abs1/1

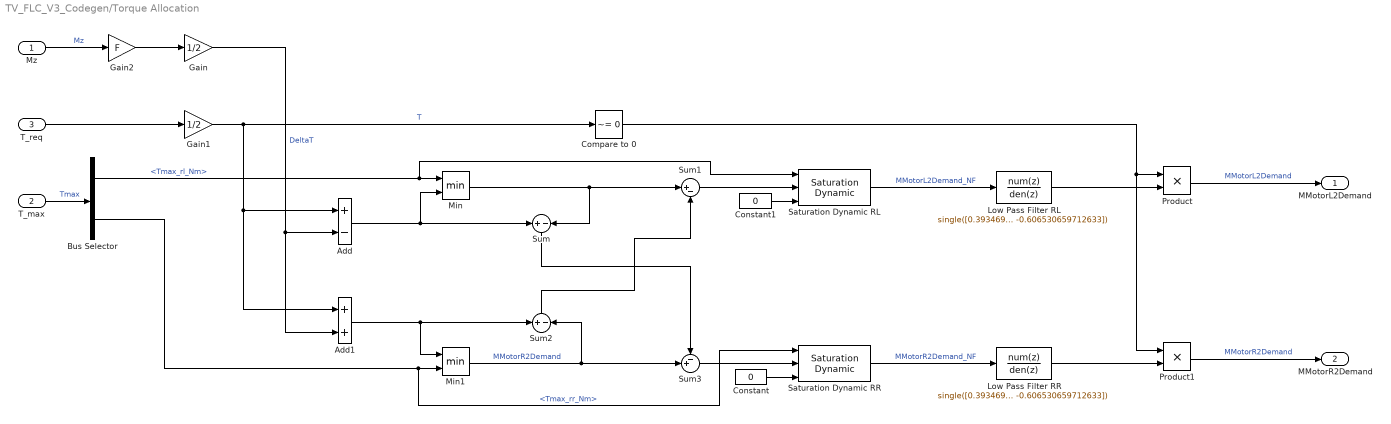
== system TV_FLC_V3_Codegen/Torque Allocation ==
  Mz : Inport
  T_max : Inport  Port=2
  T_req : Inport  Port=3
  Add : Sum  Inputs=+-
  Add1 : Sum
  Bus Selector : BusSelector  OutputSignals=Tmax_rl_Nm,Tmax_rr_Nm
  "Compare to 0 " : simulink/Logic and Bit Operations/Compare To Constant  relop=~=  const=0  OutDataTypeStr=boolean
  Constant : Constant  Value=0
  Constant1 : Constant  Value=0
  Gain : Gain  Gain=1/2
  Gain1 : Gain  Gain=1/2
  Gain2 : Gain  Gain=F
  Low Pass Filter RL : DiscreteTransferFcn  LoadFcn=dspblkCoreblockFVToolHelper(gcbh,'load');  Numerator=single([0.393469340287367])  Denominator=single([1 -0.606530659712633])
      settings: CopyFcn=dspblkCoreblockFVToolHelper(gcbh,'copy');  DeleteFcn=dspblkCoreblockFVToolHelper(gcbh,'close');  ModelCloseFcn=dspblkCoreblockFVToolHelper(gcbh,'close');  PreSaveFcn=dspblkCoreblockFVToolHelper(gcbh,'presave');  PostSaveFcn=dspblkCoreblockFVToolHelper(gcbh,'postsave');  CloseFcn=dspblkCoreblockFVToolHelper(gcbh,'close');
  Low Pass Filter RR : DiscreteTransferFcn  LoadFcn=dspblkCoreblockFVToolHelper(gcbh,'load');  Numerator=single([0.393469340287367])  Denominator=single([1 -0.606530659712633])
      settings: CopyFcn=dspblkCoreblockFVToolHelper(gcbh,'copy');  DeleteFcn=dspblkCoreblockFVToolHelper(gcbh,'close');  ModelCloseFcn=dspblkCoreblockFVToolHelper(gcbh,'close');  PreSaveFcn=dspblkCoreblockFVToolHelper(gcbh,'presave');  PostSaveFcn=dspblkCoreblockFVToolHelper(gcbh,'postsave');  CloseFcn=dspblkCoreblockFVToolHelper(gcbh,'close');
  Min : MinMax  Inputs=2
  Min1 : MinMax  Inputs=2
  Product : Product
  Product1 : Product
  Saturation Dynamic RL : sl_discontinuities/Saturation Dynamic  OutMin=[]  OutMax=[]  OutDataTypeStr=single  OutDataType=fixdt(1, 16)  OutScaling=2^-10  DoSatur=off
      settings: LibrarySourceBlock=|
      | simulink/Discontinuities/Saturation
      | Dynamic
  Saturation Dynamic RR : sl_discontinuities/Saturation Dynamic  OutMin=[]  OutMax=[]  OutDataTypeStr=single  OutDataType=fixdt(1, 16)  OutScaling=2^-10  DoSatur=off
      settings: LibrarySourceBlock=|
      | simulink/Discontinuities/Saturation
      | Dynamic
  Sum : Sum  Inputs=+|-
  Sum1 : Sum  Inputs=|+-
  Sum2 : Sum  Inputs=+|-
  Sum3 : Sum  Inputs=-+|
  MMotorL2Demand : Outport
  MMotorR2Demand : Outport  Port=2
  wires:
  Saturation Dynamic RL/1 -> Low Pass Filter RL/1  "MMotorL2Demand_NF"
  Sum3/1 -> Saturation Dynamic RR/2
  Sum1/1 -> Saturation Dynamic RL/2
  Gain2/1 -> Gain/1
  Gain/1 -> Add1/2, Add/2  "DeltaT"
  T_req/1 -> Gain1/1
  Mz/1 -> Gain2/1  "Mz"
  Min/1 -> Sum1/1, Sum/2
  Min1/1 -> Sum2/2, Sum3/2  "MMotorR2Demand"
  T_max/1 -> Bus Selector/1  "Tmax"
  Bus Selector/1 -> Saturation Dynamic RL/1, Min/1  "<Tmax_rl_Nm>"
  Bus Selector/2 -> Min1/2, Saturation Dynamic RR/1  "<Tmax_rr_Nm>"
  Add/1 -> Sum/1, Min/2
  Add1/1 -> Sum2/1, Min1/1
  Sum2/1 -> Sum1/2
  Sum/1 -> Sum3/1
  Gain1/1 -> "Compare to 0 "/1, Add1/1, Add/1  "T"
  "Compare to 0 "/1 -> Product/1, Product1/1
  Low Pass Filter RL/1 -> Product/2
  Product/1 -> MMotorL2Demand/1  "MMotorL2Demand"
  Saturation Dynamic RR/1 -> Low Pass Filter RR/1  "MMotorR2Demand_NF"
  Low Pass Filter RR/1 -> Product1/2
  Product1/1 -> MMotorR2Demand/1  "MMotorR2Demand"
  Constant/1 -> Saturation Dynamic RR/3
  Constant1/1 -> Saturation Dynamic RL/3

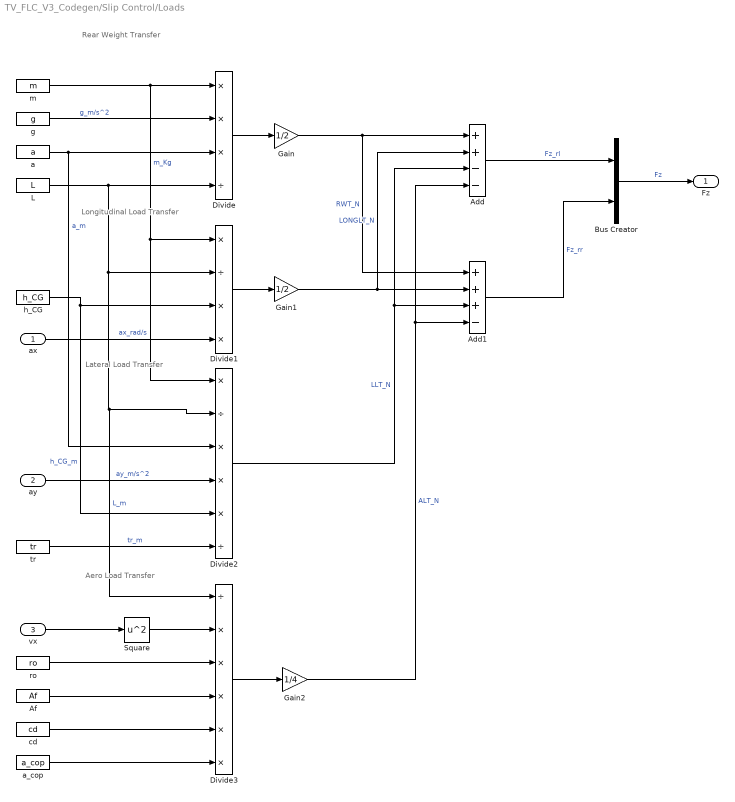
== system TV_FLC_V3_Codegen/Slip Control/Loads ==
  note: Aero Load Transfer
  note: Lateral Load Transfer
  note: Longitudinal Load Transfer
  note: Rear Weight Transfer
  ax : Inport
  ay : Inport  Port=2
  vx : Inport  Port=3
  Add : Sum  Inputs=++--
  Add1 : Sum  Inputs=+++-
  Af : Constant  Value=Af  OutDataTypeStr=single
  Bus Creator : BusCreator  Inputs=2
  Divide : Product  Inputs=***/
  Divide1 : Product  Inputs=*/**
  Divide2 : Product  Inputs=*/***/
  Divide3 : Product  Inputs=/*****
  Gain : Gain  Gain=1/2
  Gain1 : Gain  Gain=1/2
  Gain2 : Gain  Gain=1/4
  L : Constant  Value=L  OutDataTypeStr=single
  Square : Math  Operator=square
  a : Constant  Value=a  OutDataTypeStr=single
  a_cop : Constant  Value=a_cop  OutDataTypeStr=single
  cd : Constant  Value=cd  OutDataTypeStr=single
  g : Constant  Value=g  OutDataTypeStr=single
  h_CG : Constant  Value=h_CG  OutDataTypeStr=single
  m : Constant  Value=m  OutDataTypeStr=single
  ro : Constant  Value=ro  OutDataTypeStr=single
  tr : Constant  Value=tr  OutDataTypeStr=single
  Fz : Outport
  wires:
  m/1 -> Divide/1, Divide1/1, Divide2/1  "m_Kg"
  g/1 -> Divide/2  "g_m/s^2"
  a/1 -> Divide/3, Divide2/3  "a_m"
  L/1 -> Divide3/1, Divide2/2, Divide1/2, Divide/4  "L_m"
  Divide/1 -> Gain/1
  vx/1 -> Square/1
  Square/1 -> Divide3/2
  Gain/1 -> Add/1, Add1/1  "RWT_N"
  Gain2/1 -> Add/4, Add1/4  "ALT_N"
  h_CG/1 -> Divide2/5, Divide1/3  "h_CG_m"
  ax/1 -> Divide1/4  "ax_rad/s"
  Divide1/1 -> Gain1/1
  Gain1/1 -> Add/2, Add1/2  "LONGLT_N"
  ay/1 -> Divide2/4  "ay_m/s^2"
  tr/1 -> Divide2/6  "tr_m"
  Divide2/1 -> Add/3, Add1/3  "LLT_N"
  Add/1 -> Bus Creator/1  "Fz_rl"
  Add1/1 -> Bus Creator/2  "Fz_rr"
  Bus Creator/1 -> Fz/1  "Fz"
  Divide3/1 -> Gain2/1
  ro/1 -> Divide3/3
  Af/1 -> Divide3/4
  cd/1 -> Divide3/5
  a_cop/1 -> Divide3/6

== system TV_FLC_V3_Codegen/Slip Control/Maximum Torque Allowed ==
  Fz : Inport
  kappa_rl : Inport  Port=2
  kappa_rr : Inport  Port=3
  Bus Creator : BusCreator  Inputs=2
  Bus Selector : BusSelector  OutputSignals=Fz_rl,Fz_rr
  Slip Correction Left : Subsystem
  Slip Correction Right : Subsystem
  Tmax : Outport  OutDataTypeStr=single
  Out Bus Element : Outport  Port=2  PortName=Debug  Element=PID_rl
  Out Bus Element1 : Outport  Port=2  PortName=Debug  Element=PID_rr
  wires:
  Bus Creator/1 -> Tmax/1
  Bus Selector/2 -> Slip Correction Right/1(Fz_rl)  "<Fz_rr>"
  Bus Selector/1 -> Slip Correction Left/2(Fz_rl)  "<Fz_rl>"
  Fz/1 -> Bus Selector/1
  kappa_rr/1 -> Slip Correction Right/2(kappa_rr)
  kappa_rl/1 -> Slip Correction Left/1(kappa_rl)
  Slip Correction Left/2(Tmax_rl) -> Bus Creator/1  "Tmax_rl_Nm"
  Slip Correction Right/1(Tmax_rr) -> Bus Creator/2  "Tmax_rr_Nm"
  Slip Correction Left/1(Debug) -> Out Bus Element/1
  Slip Correction Right/2(Debug) -> Out Bus Element1/1

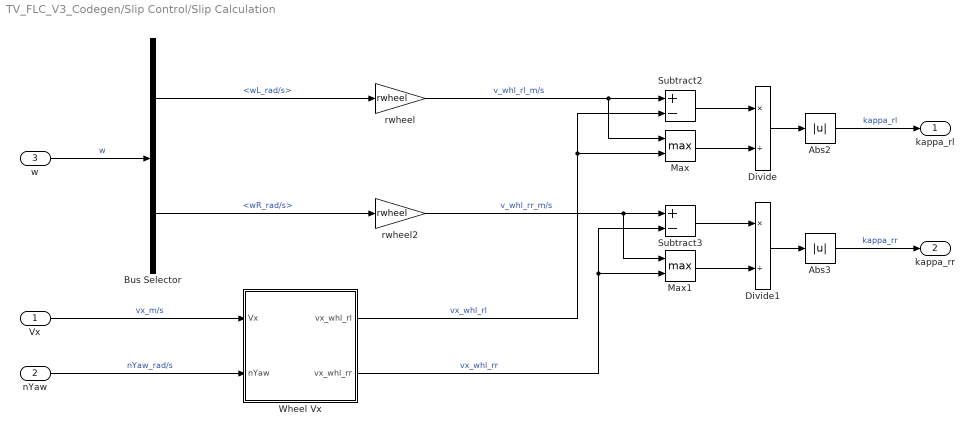
== system TV_FLC_V3_Codegen/Slip Control/Slip Calculation ==
  Vx : Inport
  nYaw : Inport  Port=2
  w : Inport  Port=3
  Abs2 : Abs  SaturateOnIntegerOverflow=off
  Abs3 : Abs  SaturateOnIntegerOverflow=off
  Bus Selector : BusSelector  OutputSignals=wL_rad/s,wR_rad/s
  Divide : Product  Inputs=*/
  Divide1 : Product  Inputs=*/
  Max : MinMax  Function=max  Inputs=2
  Max1 : MinMax  Function=max  Inputs=2
  Subtract2 : Sum  Inputs=+-
  Subtract3 : Sum  Inputs=+-
  Wheel Vx : Subsystem
  rwheel : Gain  Gain=rwheel
  rwheel2 : Gain  Gain=rwheel
  kappa_rl : Outport
  kappa_rr : Outport  Port=2
  wires:
  Bus Selector/1 -> rwheel/1  "<wL_rad/s>"
  Bus Selector/2 -> rwheel2/1  "<wR_rad/s>"
  Vx/1 -> Wheel Vx/1(Vx)  "vx_m/s"
  w/1 -> Bus Selector/1  "w"
  rwheel/1 -> Max/1, Subtract2/1  "v_whl_rl_m/s"
  rwheel2/1 -> Max1/1, Subtract3/1  "v_whl_rr_m/s"
  nYaw/1 -> Wheel Vx/2(nYaw)  "nYaw_rad/s"
  Abs3/1 -> kappa_rr/1  "kappa_rr"
  Wheel Vx/1(vx_whl_rl) -> Subtract2/2, Max/2  "vx_whl_rl"
  Abs2/1 -> kappa_rl/1  "kappa_rl"
  Subtract2/1 -> Divide/1
  Wheel Vx/2(vx_whl_rr) -> Subtract3/2, Max1/2  "vx_whl_rr"
  Subtract3/1 -> Divide1/1
  Divide/1 -> Abs2/1
  Max/1 -> Divide/2
  Divide1/1 -> Abs3/1
  Max1/1 -> Divide1/2

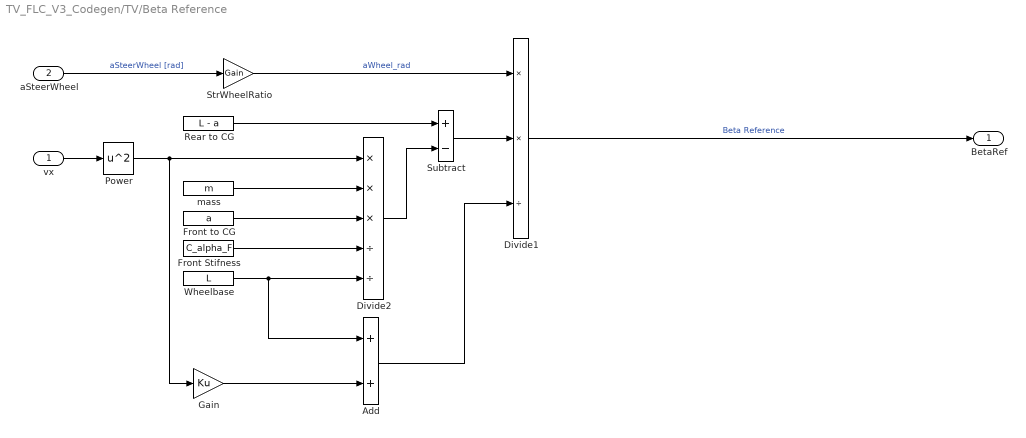
== system TV_FLC_V3_Codegen/TV/Beta Reference ==
  vx : Inport
  aSteerWheel : Inport  Port=2
  Add : Sum
  Divide1 : Product  Inputs=**/
  Divide2 : Product  Inputs=***//
  Front Stifness : Constant  Value=C_alpha_F  OutDataTypeStr=single
  Front to CG : Constant  Value=a  OutDataTypeStr=single
  Gain : Gain  Gain=Ku  ParamDataTypeStr=single
  Power : Math  Operator=square
  Rear to CG : Constant  Value=L - a  OutDataTypeStr=single
  StrWheelRatio : Gain  Gain=Gain
  Subtract : Sum  Inputs=+-
  Wheelbase : Constant  Value=L  OutDataTypeStr=single
  mass : Constant  Value=m  OutDataTypeStr=single
  BetaRef : Outport
  wires:
  StrWheelRatio/1 -> Divide1/1  "aWheel_rad"
  Add/1 -> Divide1/3
  Gain/1 -> Add/2
  Power/1 -> Gain/1, Divide2/1
  Divide1/1 -> BetaRef/1  "Beta Reference"
  vx/1 -> Power/1
  aSteerWheel/1 -> StrWheelRatio/1  "aSteerWheel [rad]"
  Wheelbase/1 -> Add/1, Divide2/5
  Front Stifness/1 -> Divide2/4
  mass/1 -> Divide2/2
  Front to CG/1 -> Divide2/3
  Rear to CG/1 -> Subtract/1
  Divide2/1 -> Subtract/2
  Subtract/1 -> Divide1/2

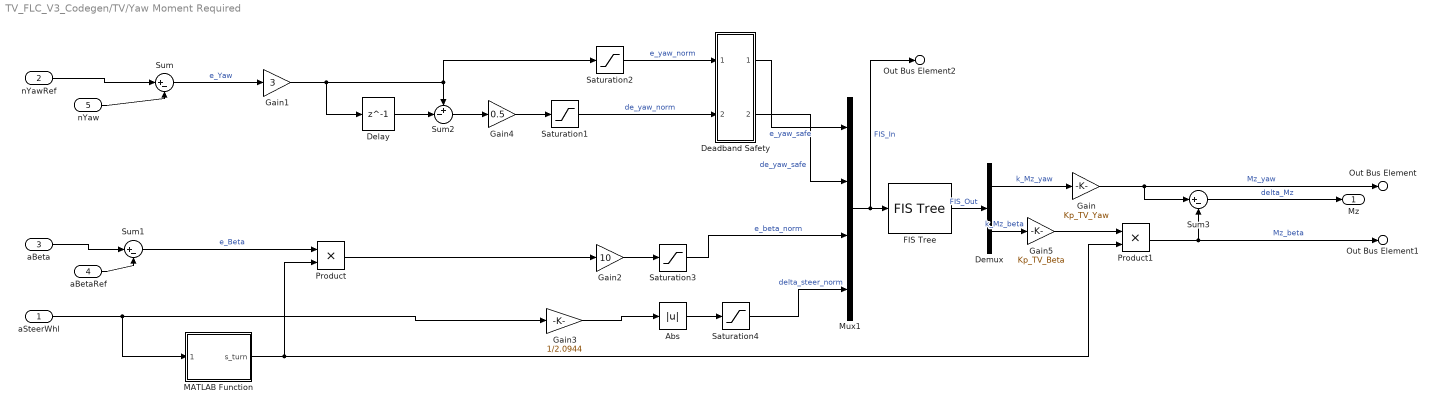
== system TV_FLC_V3_Codegen/TV/Yaw Moment Required ==
  aSteerWhl : Inport  OutDataTypeStr=single
  nYawRef : Inport  Port=2  OutDataTypeStr=single
  aBeta : Inport  Port=3  OutDataTypeStr=single
  aBetaRef : Inport  Port=4  OutDataTypeStr=single
  nYaw : Inport  Port=5  OutDataTypeStr=single
  Abs : Abs  SaturateOnIntegerOverflow=off
  Deadband Safety : Subsystem
  Delay : Delay  DelayLength=1  InputProcessing=Columns as channels (frame based)
  Demux : Demux  Outputs=2
  FIS Tree : fuzblock/FIS Tree  FIS=FIS_DYC_3  OutputSampleNumber=101  DataType=single  SimulateUsing=Code generation  OutOfRangeInputValueMessage=warning  NoRuleFiredMessage=warning  EmptyOutputFuzzySetMessage=warning
  Gain : Gain  Gain=Kp_TV_Yaw  OutDataTypeStr=single
  Gain1 : Gain  Gain=3
  Gain2 : Gain  Gain=10  OutDataTypeStr=single
  Gain3 : Gain  Gain=1/2.0944  OutDataTypeStr=single
  Gain4 : Gain  Gain=0.5
  Gain5 : Gain  Gain=Kp_TV_Beta  OutDataTypeStr=single
  MATLAB Function : MATLAB Function  TreatAsAtomicUnit=on  mask{delta_th=Slip_Steer_th/2}
      mask prompts: delta_th "Steering Th"
  Mux1 : Mux
  Product : Product
  Product1 : Product
  Saturation1 : Saturate  UpperLimit=1  LowerLimit=-1
  Saturation2 : Saturate  UpperLimit=1  LowerLimit=-1
  Saturation3 : Saturate  UpperLimit=1  LowerLimit=-1  ZeroCross=off
  Saturation4 : Saturate  UpperLimit=1  LowerLimit=0  ZeroCross=off
  Sum : Sum  Inputs=|+-
  Sum1 : Sum  Inputs=|+-
  Sum2 : Sum  Inputs=+-|
  Sum3 : Sum  Inputs=|+-  OutDataTypeStr=Inherit: Same as first input
  Mz : Outport  OutDataTypeStr=single
  Out Bus Element : Outport  Port=2  PortName=Debug  Element=Mz_yaw
  Out Bus Element1 : Outport  Port=2  PortName=Debug  Element=Mz_Beta
  Out Bus Element2 : Outport  Port=2  PortName=Debug  Element=FIS_In
  wires:
  Sum/1 -> Gain1/1  "e_Yaw"
  nYaw/1 -> Sum/2
  nYawRef/1 -> Sum/1
  FIS Tree/1 -> Demux/1  "FIS_Out"
  Gain/1 -> Out Bus Element/1, Sum3/1  "Mz_yaw"
  Delay/1 -> Sum2/2
  Sum2/1 -> Gain4/1
  Mux1/1 -> Out Bus Element2/1, FIS Tree/1  "FIS_In"
  Sum1/1 -> Product/1  "e_Beta"
  aBeta/1 -> Sum1/1
  aBetaRef/1 -> Sum1/2
  aSteerWhl/1 -> Gain3/1, MATLAB Function/1(delta_SW)
  Gain1/1 -> Delay/1, Sum2/1, Saturation2/1
  Gain2/1 -> Saturation3/1
  Gain3/1 -> Abs/1
  Saturation3/1 -> Mux1/3  "e_beta_norm"
  Saturation4/1 -> Mux1/4  "delta_steer_norm"
  Gain4/1 -> Saturation1/1
  MATLAB Function/1(s_turn) -> Product/2, Product1/2
  Product/1 -> Gain2/1
  Demux/1 -> Gain/1  "k_Mz_yaw"
  Demux/2 -> Gain5/1  "k_Mz_beta"
  Sum3/1 -> Mz/1  "delta_Mz"
  Gain5/1 -> Product1/1
  Product1/1 -> Out Bus Element1/1, Sum3/2  "Mz_beta"
  Abs/1 -> Saturation4/1
  Saturation2/1 -> Deadband Safety/1(e_yaw_norm)  "e_yaw_norm"
  Saturation1/1 -> Deadband Safety/2(de_yaw_norm)  "de_yaw_norm"
  Deadband Safety/1(e_yaw_safe) -> Mux1/1  "e_yaw_safe"
  Deadband Safety/2(de_yaw_safe) -> Mux1/2  "de_yaw_safe"

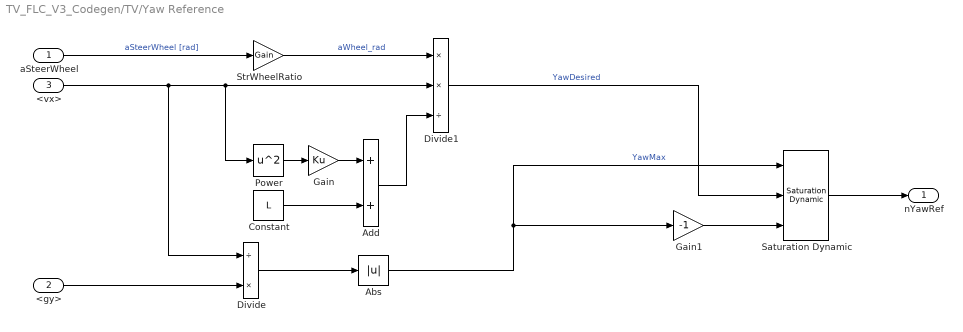
== system TV_FLC_V3_Codegen/TV/Yaw Reference ==
  aSteerWheel : Inport
  <gy> : Inport  Port=2
  <vx> : Inport  Port=3
  Abs : Abs  SaturateOnIntegerOverflow=off
  Add : Sum
  Constant : Constant  Value=L  OutDataTypeStr=single
  Divide : Product  Inputs=/*
  Divide1 : Product  Inputs=**/
  Gain : Gain  Gain=Ku
  Gain1 : Gain  Gain=-1
  Power : Math  Operator=square
  Saturation Dynamic : sl_discontinuities/Saturation Dynamic  OutMin=[]  OutMax=[]  OutDataTypeStr=Inherit: Same as second input  OutDataType=fixdt(1, 16)  OutScaling=2^-10  DoSatur=off
  StrWheelRatio : Gain  Gain=Gain
  nYawRef : Outport
  wires:
  StrWheelRatio/1 -> Divide1/1  "aWheel_rad"
  aSteerWheel/1 -> StrWheelRatio/1  "aSteerWheel [rad]"
  <vx>/1 -> Divide1/2, Power/1, Divide/1
  <gy>/1 -> Divide/2
  Divide/1 -> Abs/1
  Saturation Dynamic/1 -> nYawRef/1
  Abs/1 -> Saturation Dynamic/1, Gain1/1  "YawMax"
  Gain1/1 -> Saturation Dynamic/3
  Divide1/1 -> Saturation Dynamic/2  "YawDesired"
  Power/1 -> Gain/1
  Gain/1 -> Add/1
  Constant/1 -> Add/2
  Add/1 -> Divide1/3

== system TV_FLC_V3_Codegen/Slip Control/Maximum Torque Allowed/Slip Correction Left ==
  kappa_rl : Inport  OutDataTypeStr=single
  Fz_rl : Inport  Port=2  OutDataTypeStr=single
  1-D Lookup Table : Lookup_n-D  NumberOfTableDimensions=1  BreakpointsForDimension1=Load_Ref  Table=Slip_Ref  ExtrapMethod=Clip  UseLastTableValue=on  InternalRulePriority=Speed  RndMeth=Simplest
  PID Controller : slpidlib/PID Controller  Controller=PID  Form=Parallel  TimeDomain=Discrete-time  UseExternalTs=off  SampleTime=0.003  IntegratorMethod=Forward Euler  FilterMethod=Forward Euler  ControllerParametersSource=internal  P=Slip_Ctrl_Kp  I=Slip_Ctrl_Ki  UseKiTs=off  D=Slip_Ctrl_Kd  UseExternalDerivativeSource=off  N=Slip_Ctrl_Kn  UseFilter=on  TunerSelectOption=Transfer Function Based (PID Tuner App)  InitialConditionSource=internal  InitialConditionForIntegrator=Tmax  InitialConditionForFilter=0  DifferentiatorICPrevScaledInput=Tmax  ExternalReset=none  TrackingMode=off  Kt=1  LimitOutput=on  SatLimitsSource=internal  UpperSaturationLimit=Tmax  LowerSaturationLimit=0  LinearizeAsGain=on  AntiWindupMode=clamping  Kb=1  LimitIntegrator=off  UpperIntegratorSaturationLimit=inf  LowerIntegratorSaturationLimit=-inf  POutMin=[]  POutMax=[]  IOutMin=[]  IOutMax=[]  DOutMin=[]  DOutMax=[]  NOutMin=[]  NOutMax=[]  SumOutMin=[]  SumOutMax=[]  SaturationOutMin=[]  SaturationOutMax=[]  PParamMin=[]  PParamMax=[]  IParamMin=[]  IParamMax=[]  DParamMin=[]  DParamMax=[]  NParamMin=[]  NParamMax=[]  KbParamMin=[]  KbParamMax=[]  KtParamMin=[]  KtParamMax=[]  KbOutMin=[]  KbOutMax=[]  KtOutMin=[]  KtOutMax=[]  IntegratorOutMin=[]  IntegratorOutMax=[]  FilterOutMin=[]  FilterOutMax=[]  SumI1OutMin=[]  SumI1OutMax=[]  SumI2OutMin=[]  SumI2OutMax=[]  SumI3OutMin=[]  SumI3OutMax=[]  SumI4OutMin=[]  SumI4OutMax=[]  SumDOutMin=[]  SumDOutMax=[]  DifferentiatorOutMin=[]  DifferentiatorOutMax=[]  FilterDiffOutCoefMin=[]  FilterDiffOutCoefMax=[]  ReciprocalOutMin=[]  ReciprocalOutMax=[]  SumDenOutMin=[]  SumDenOutMax=[]  SumNumOutMin=[]  SumNumOutMax=[]  DivideOutMin=[]  DivideOutMax=[]  UdiffTsProdOutMin=[]  UdiffTsProdOutMax=[]  NTsProdOutMin=[]  NTsProdOutMax=[]  UintegralTsProdOutMin=[]  UintegralTsProdOutMax=[]  UngainTsProdOutMin=[]  UngainTsProdOutMax=[]  ClampingZeroOutDataTypeStr=Inherit: Inherit via back propagation  ClampingZeroOutMin=[]  ClampingZeroOutMax=[]  FilterDenConstantOutDataTypeStr=Inherit: Inherit via back propagation  FilterDenConstantOutMin=[]  FilterDenConstantOutMax=[]  PCopyOutDataTypeStr=Inherit: Inherit via back propagation  PCopyOutMin=[]  PCopyOutMax=[]  NCopyOutDataTypeStr=Inherit: Inherit via back propagation  NCopyOutMin=[]  NCopyOutMax=[]  IntegratorContinuousStateAttributes=''  IntegratorStateMustResolveToSignalObject=off  IntegratorRTWStateStorageClass=Auto  FilterContinuousStateAttributes=''  FilterStateMustResolveToSignalObject=off  FilterRTWStateStorageClass=Auto  ParallelPVariant=InternalParameters  IdealPVariant=Disabled  IVariant=InternalParameters  DVariant=InternalParameters  IntegratorVariant=Discrete  SatVariant=Enabled  AWVariant=DiscClampingParallel  PCopyVariant=Disabled  TRVariant=Disabled  FdbkBlocksVariant=Forward  IdealPFdbkVariant=Disabled  SatFdbkVariant=Disabled  DerivativeFilterVariant=ForwardEulerFilter  NVariant=InternalParameters  NCopyVariant=Disabled  FilterICVariant=InternalICsFilter  IntegratorICVariant=InternalICs  ExternalResetVariant=Disabled  TRSumVariant=Passthrough  SumFdbkVariant=Disabled  SumVariant=Sum_PID  TsampFilterVariant=InternalTs  TsampNgainVariant=Passthrough  TsampIntegralVariant=Disabled_SignalSpec  ExternalSaturationOutDataTypeStr=Inherit: Same as second input  DerivativeSourceVariant=ErrorSignal  PreIntVariant=InternalPreInt
  Sum : Sum  Inputs=|+-
  Out Bus Element : Outport  PortName=Debug  Element=kappa_rl_ref
  Tmax_rl : Outport  Port=2
  wires:
  PID Controller/1 -> Tmax_rl/1  "Tmax_rl_Nm"
  kappa_rl/1 -> Sum/2  "kappa_rl"
  1-D Lookup Table/1 -> Out Bus Element/1, Sum/1  "kappa_ref"
  Sum/1 -> PID Controller/1  "e"
  Fz_rl/1 -> 1-D Lookup Table/1  "Fz_rl_N"
